simulink model "task6"  (R2024b)
settings: Solver=VariableStepAuto  StartTime=0.0  StopTime=10.0  RelTol=1e-3
settings Model: Creator=33657  LastModifiedBy=33657

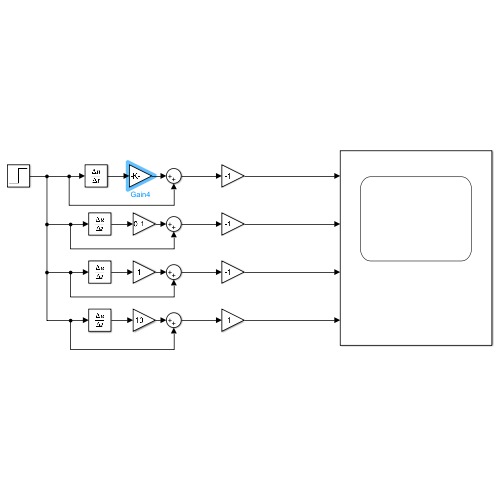
[thumbnail: Simulink's stored preview of the top-level diagram]
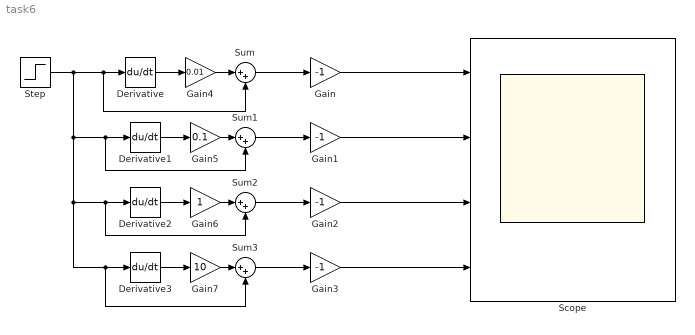
== system task6 ==
  Derivative{,1..3} (4 alike) : Derivative
  Gain{,1..3} (4 alike) : Gain  Gain=-1
  Gain4 : Gain  Gain=0.01
  Gain5 : Gain  Gain=0.1
  Gain6 : Gain
  Gain7 : Gain  Gain=10
  Scope : Scope  NumInputPorts=4
  Step : Step  SampleTime=0
  Sum{,1..3} (4 alike) : Sum  Inputs=|++
  wires:
  Sum/1 -> Gain/1
  Gain/1 -> Scope/1
  Step/1 -> Derivative/1, Sum/2, Derivative1/1, Sum1/2, Derivative2/1, Sum2/2, Derivative3/1, Sum3/2
  Sum1/1 -> Gain1/1
  Sum2/1 -> Gain2/1
  Sum3/1 -> Gain3/1
  Gain1/1 -> Scope/2
  Gain2/1 -> Scope/3
  Gain3/1 -> Scope/4
  Gain4/1 -> Sum/1
  Derivative/1 -> Gain4/1
  Derivative1/1 -> Gain5/1
  Derivative2/1 -> Gain6/1
  Derivative3/1 -> Gain7/1
  Gain5/1 -> Sum1/1
  Gain7/1 -> Sum3/1
  Gain6/1 -> Sum2/1
